simulink model "control_cinmatica"  (R2025b)
settings: Solver=VariableStepAuto  StartTime=0.0  StopTime=10.0  RelTol=1e-3
settings Model: Creator=dssr2  LastModifiedBy=dssr2

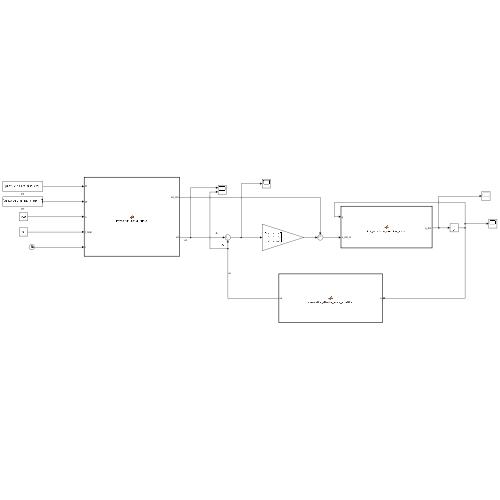
[thumbnail: Simulink's stored preview of the top-level diagram]
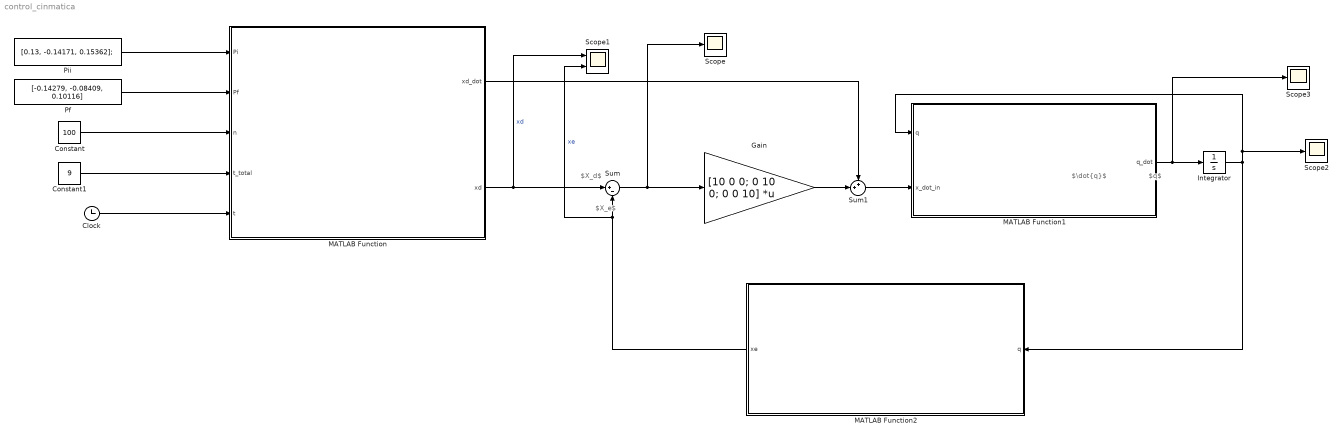
== system control_cinmatica ==
  note: $X_e$
  note: $X_d$
  note: $q$
  note: $\dot{q}$
  Clock : Clock
  Constant : Constant  Value=100
  Constant1 : Constant  Value=9
  Gain : Gain  Gain=[10 0 0; 0 10 0; 0 0 10]  Multiplication=Matrix(K*u)
  Integrator : Integrator
  MATLAB Function : MATLAB Function  TreatAsAtomicUnit=on
  MATLAB Function1 : MATLAB Function  TreatAsAtomicUnit=on
  MATLAB Function2 : MATLAB Function  TreatAsAtomicUnit=on
  Pf : Constant  Value=[-0.14279, -0.08409, 0.10116]
  Pii : Constant  Value=[0.13, -0.14171, 0.15362];
  Scope : Scope
      settings: ActiveDisplayYMinimum=-0.07072708816866996  ActiveDisplayYMaximum=0.010772764827806407
  Scope1 : Scope  NumInputPorts=2
      settings: ActiveDisplayYMinimum=-0.292125  ActiveDisplayYMaximum=0.399125
  Scope2 : Scope
      settings: ActiveDisplayYMinimum=-0.35632844057715568  ActiveDisplayYMaximum=0.19452849879069517  DataLoggingVariableName=ScopeData2
  Scope3 : Scope
      settings: ActiveDisplayYMinimum=-0.19444388468459015  ActiveDisplayYMaximum=0.10301630386455493  DataLoggingVariableName=ScopeData3
  Sum : Sum  Inputs=|+-
  Sum1 : Sum  Inputs=++|
  wires:
  MATLAB Function1/1(q_dot) -> Scope3/1, Integrator/1
  Integrator/1 -> MATLAB Function2/1(q), Scope2/1, MATLAB Function1/1(q)
  MATLAB Function2/1(xe) -> Scope1/2, Sum/2  "xe"
  Clock/1 -> MATLAB Function/5(t)
  Sum1/1 -> MATLAB Function1/2(x_dot_in)
  Constant/1 -> MATLAB Function/3(n)
  Gain/1 -> Sum1/2
  Pf/1 -> MATLAB Function/2(Pf)
  Sum/1 -> Scope/1, Gain/1
  Constant1/1 -> MATLAB Function/4(t_total)
  MATLAB Function/2(xd) -> Scope1/1, Sum/1  "xd"
  MATLAB Function/1(xd_dot) -> Sum1/1
  Pii/1 -> MATLAB Function/1(Pi)

== matlab function control_cinmatica/MATLAB Function1 ==
  data: q input size=3; q_dot output; x_dot_in input
function q_dot = inv_jacobiano_analitico_scara(q, x_dot_in)
% INV_JACOBIANO_ANALITICO_SCARA
% Entradas:
%   q        : Posiciones articulares [th1; th2; d3] (3x1)
%   x_dot_in : Velocidad cartesiana de entrada (xd_dot + K*e) (3x1)
%
% Salida:
%   q_dot    : Velocidad articular [th1_dot; th2_dot; d3_dot] (3x1)

    th1 = q(1);
    th2 = q(2);
    % d3  = q(3); % No interviene directamente en la derivada del plano XY

    % Parámetros geométricos del SCARA
    a1 = 0.13;
    a2 = 0.13571 + 0.006;

    % Ángulo equivalente del segundo eslabón según la convención DH usada
    th12 = th1 + (th2 - (pi/2));

    % --- Construcción del Jacobiano Analítico Ja(q) (3x3) ---
    % Fila 1: dx/d_th1, dx/d_th2, dx/d_d3
    J11 = -a1*sin(th1) - a2*sin(th12);
    J12 = -a2*sin(th12);
    J13 = 0;

    % Fila 2: dy/d_th1, dy/d_th2, dy/d_d3
    J21 =  a1*cos(th1) + a2*cos(th12);
    J22 =  a2*cos(th12);
    J23 = 0;

    % Fila 3: dz/d_th1, dz/d_th2, dz/d_d3
    J31 = 0;
    J32 = 0;
    J33 = -1;  % Pz = d1 + d2 - d3  ->  d(Pz)/d(d3) = -1

    % Matriz Jacobiana Analítica 3x3
    Ja = [J11, J12, J13;
          J21, J22, J23;
          J31, J32, J33];

    % Inversa de la matriz Jacobiana analítica para obtener las velocidades articulares
    q_dot = pinv(Ja) * x_dot_in;
end

== matlab function control_cinmatica/MATLAB Function ==
  settings: updateMethod=DISCRETE
  data: xd_dot output; xd output; Pi input; Pf input; n input; t_total input; t input
function [xd_dot, xd] = trayectoria_scara_punto(Pi, Pf, n, t_total, t)
%#codegen
% TRAYECTORIA_SCARA_PUNTO  Referencia (xd, xd_dot) planeada con el Jacobiano inverso.
%
%   En vez de interpolar la recta, la trayectoria se PLANEA integrando
%       q_dot = inv(Jv(q)) * v_e,      q(k+1) = q(k) + q_dot*dt
%   desde q0 = cinematica_inversa(Pi), igual que el script de planeacion. La posicion
%   deseada es la cinematica directa de esa q planeada: xd = k(q_plan).
%   Se calcula UNA vez (variables persistentes) y despues solo se consulta.
%
%   Entradas:
%     Pi, Pf   : puntos inicial y final [x y z] en m
%     n        : numero de pasos de la planeacion
%     t_total  : duracion total [s]
%     t        : TIEMPO actual de simulacion [s]  (conectar el bloque Clock aqui;
%                antes esta entrada se llamaba paso_actual y se leia como indice)
%   Salidas:
%     xd       : posicion deseada [x; y; z]   (interpolada linealmente entre muestras)
%     xd_dot   : velocidad deseada [vx; vy; vz] (constante; 0 al llegar)

    NMAX = 3000;                    % tamano maximo reservado para la planeacion
    USAR_PUNTO_MEDIO = false;       % false: Euler adelante (como el script). true: mas exacto

    persistent Pplan Pi_p Pf_p n_p T_p listo
    if isempty(listo)
        Pplan = zeros(3, NMAX+1);
        Pi_p = zeros(1,3);  Pf_p = zeros(1,3);  n_p = 0;  T_p = 0;
        listo = false;
    end

    Pi = Pi(:)';  Pf = Pf(:)';
    n = min(max(round(n), 1), NMAX);
    T = max(t_total, eps);

    % Planear de nuevo solo si cambia algun dato
    if ~listo || any(Pi ~= Pi_p) || any(Pf ~= Pf_p) || n ~= n_p || T ~= T_p
        Pplan = planear_con_jacobiano(Pi, Pf, n, T, NMAX, USAR_PUNTO_MEDIO);
        Pi_p = Pi;  Pf_p = Pf;  n_p = n;  T_p = T;  listo = true;
    end

    % Consulta en el instante t (interpolacion lineal entre las muestras planeadas)
    dt = T / n;
    k  = min(max(t, 0), T) / dt;
    i0 = min(floor(k), n-1);
    f  = k - i0;
    xd = (1-f)*Pplan(:, i0+1) + f*Pplan(:, i0+2);

    v_e = ((Pf - Pi) / T)';
    if t >= T
        xd_dot = zeros(3,1);        % se detiene al llegar al final
    else
        xd_dot = v_e;
    end
end


%% ------------- Planeacion con Jacobiano inverso -------------
function P = planear_con_jacobiano(Pi, Pf, n, T, NMAX, usar_punto_medio)
    P  = zeros(3, NMAX+1);
    dt = T / n;
    v_e = ((Pf - Pi) / T)';                 % velocidad cartesiana constante 3x1

    q = cinematica_inversa_ar(Pi(1), Pi(2), Pi(3));
    [~, Px, Py, Pz] = cinematica(q(1), q(2), q(3));
    P(:,1) = [Px; Py; Pz];

    for i = 1:n
        [~, ~, ~, ~, J] = cinematica(q(1), q(2), q(3));
        q_dot = resolver(J(1:3,:), v_e);                 % q_dot = inv(Jv) * v_e
        if usar_punto_medio
            qm = q + 0.5*dt*q_dot;
            [~, ~, ~, ~, Jm] = cinematica(qm(1), qm(2), qm(3));
            q_dot = resolver(Jm(1:3,:), v_e);
        end
        q = q + q_dot*dt;                                % Euler hacia adelante
        [~, Px, Py, Pz] = cinematica(q(1), q(2), q(3));
        P(:,i+1) = [Px; Py; Pz];
    end
end

function qd = resolver(Jv, v)
    if abs(det(Jv)) < 1e-8
        qd = zeros(3,1);                    % singularidad: no se mueve
    else
        qd = Jv \ v;
    end
end


%% ------------- Cinematica directa y Jacobiano -------------
function [T, Px, Py, Pz, J] = cinematica(th1, th2, d3)
    d1 = 0.15;   d2 = 0.06;
    a1 = 0.13;   a2 = 0.13571 + 0.006;

    A1 = tqi(th1,        d1, 0,  a1);
    A2 = tqi(th2 - pi/2, d2, pi, a2);
    A3 = tqi(0,          d3, 0,  0);

    T1 = A1;  T2 = A1*A2;  T3 = T2*A3;
    T = T3;
    Px = T(1,4);  Py = T(2,4);  Pz = T(3,4);

    z0 = [0;0;1];     p0 = [0;0;0];
    z1 = T1(1:3,3);   p1 = T1(1:3,4);
    z2 = T2(1:3,3);
    pe = T3(1:3,4);

    J = [cross(z0, pe-p0), cross(z1, pe-p1), z2;
         z0,               z1,               [0;0;0]];
end

function Tq = tqi(tht, d, alp, a)
    ct = cos(tht);  st = sin(tht);
    ca = cos(alp);  sa = sin(alp);
    Tq = [ct, -st*ca,  st*sa, a*ct;
          st,  ct*ca, -ct*sa, a*st;
          0,   sa,     ca,    d;
          0,   0,      0,     1];
end

%% ------------- Cinematica inversa (rama 'ar', solo condicion inicial) -------------
function q = cinematica_inversa_ar(Px, Py, Pz)
    a1 = 0.13;  a2 = 0.13571 + 0.006;
    d1 = 0.15;  d2 = 0.06;

    aph = atan2(Py, Px);
    d   = hypot(Px, Py);

    cosB   = max(-1, min(1, (d^2 + a1^2 - a2^2)/(2*d*a1)));
    cosphi = max(-1, min(1, (a1^2 + a2^2 - d^2)/(2*a1*a2)));
    B   = acos(cosB);
    phi = acos(cosphi);

    th1 = atan2(sin(aph + B), cos(aph + B));
    th2 = atan2(sin(phi - pi/2), cos(phi - pi/2));
    d3  = (d1 + d2) - Pz;             % consistente con la cinematica directa: Pz = d1 + d2 - d3

    q = [th1; th2; d3];
end

== matlab function control_cinmatica/MATLAB Function2 ==
  data: q input; xe output
function xe = cinematica_directa_scara_analitica(q)
    th1 = q(1);
    th2 = q(2);
    d3  = q(3);

    a1 = 0.13;
    a2 = 0.13571 + 0.006;
    d1 = 0.15;
    d2 = 0.06;

    th12 = th1 + th2 - (pi/2);

    x = a1*cos(th1) + a2*cos(th12);
    y = a1*sin(th1) + a2*sin(th12);
    z = (d1 + d2) - d3;

    xe = [x; y; z];
end
